simulink model "SAcell"  (R2023b)
settings: Solver=ode1  StartTime=0.0  StopTime=5000  FixedStep=0.1  RelTol=1e-3  EnableMultiTasking=on
model workspace: external: MAT-File SA.mat (data not in the file)
values from neighbouring files (symbols this model uses):
  bcl = 1500    [BH.mat]    (also in CN.mat; SA.mat = 814)
  erp = 108    [BH.mat]    (also in CN.mat = 214; SA.mat = 161.5)
  f = 0    [BH.mat]    (also in CN.mat = 0.8; SA.mat = 0.1)
  h = 0    [BH.mat]    (also in CN.mat = 0.2; Plottrace.m = gca; SA.mat = 0.2; plotCells.m = gca)
  hr = 0.1    [BH.mat]    (also in CN.mat; SA.mat)
  hs = 35    [BH.mat]    (also in CN.mat; SA.mat)
  j = 2    [BH.mat]    (also in CN.mat = 0; SA.mat = 0)
  m = 1    [BH.mat]    (also in CN.mat; SA.mat; plotCells.m; plotCells_second.m)
  r = 0.5    [BH.mat]    (also in CN.mat; SA.mat)
  s = 5    [BH.mat]    (also in CN.mat; SA.mat; plotCells.m = [4 8 9 10 11]; plotCells_second.m = [4 8 9 10 11])
  Vh = -15    [BH.mat]    (also in CN.mat = -4; SA.mat = -4)
libraries: Libs x1
settings Model: PauseTimes=18000  Creator=wai484  LastModifiedBy=wai484
settings SolverCC: AlgebraicLoopSolver=TrustRegion
settings DataIOCC: LimitDataPoints=on  SaveFormat=Array  ReturnWorkspaceOutputs=off
settings OptimizationCC: LifeSpan=inf
settings DebuggingCC: SolverPrmCheckMsg=warning  UnconnectedInputMsg=warning  UnconnectedOutputMsg=warning  UnconnectedLineMsg=warning  SFUnexpectedBacktrackingDiag=warning  SFNoUnconditionalDefaultTransitionDiag=warning  SFExecutionAtInitializationDiag=none  ArithmeticOperatorsInVariantConditions=warning
settings HardwareCC: ProdBitPerPointer=32  ProdBitPerSizeT=32  ProdBitPerPtrDiffT=32  ProdLargestAtomicFloat=None  ProdIntDivRoundTo=Undefined  ProdEndianess=Unspecified  ProdWordSize=32  ProdHWDeviceType=32-bit Generic
settings ModelReferenceCC: EnableRefExpFcnMdlSchedulingChecks=on  PropagateSignalLabelsOutOfModel=off
settings SFSimCC: SimUseLocalCustomCode=off  CustomCodeUndefinedFunction=UseInterfaceOnly
settings RTWCC: RTWUseLocalCustomCode=off
settings CodeAppCC: StateflowObjectComments=on
settings GRTTargetCC: TargetLangStandard=C89/C90 (ANSI)
settings ConfigComp: CovMetricSettings=dw  CovSaveCumulativeToWorkspaceVar=on  CovSaveSingleToWorkspaceVar=on  CovExternalEMLEnable=off  CovSFcnEnable=off

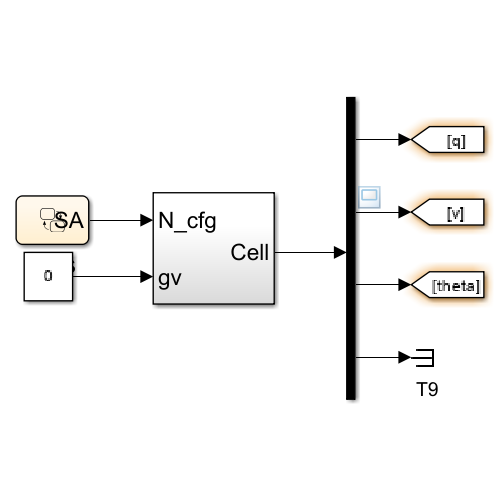
[thumbnail: Simulink's stored preview of the top-level diagram]
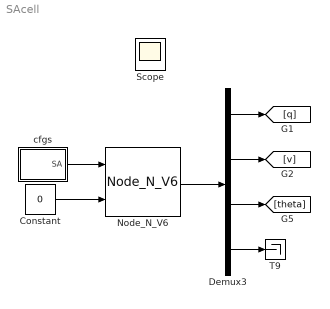
== system SAcell ==
  Constant : Constant  Value=0
  Demux3 : Demux  Outputs=[1, 1, 1,2]
  Node_N_V6 : Libs/Node_N_V6  SystemSampleTime=-1  VariantActivationTime=update diagram  AllowFlexibleInterface=on  Latency=0  AutoFrameSizeCalculation=off
  T9 : Terminator
  cfgs : Stateflow chart  TreatAsAtomicUnit=on
  Scope : Scope
  wires:
  Node_N_V6/1 -> Demux3/1
  Demux3/4 -> T9/1
  Demux3/1 -> [q]
  Demux3/2 -> [v]
  Demux3/3 -> [theta]
  Constant/1 -> Node_N_V6/2
  cfgs/1(SA) -> Node_N_V6/1

== stateflow chart SAcell/cfgs ==
  settings: executeAtInitialization=1
  state Ini
  (default) -> Ini : {SA=auto;}
  data: erp parameter; Vh parameter; hr parameter; hs parameter; m parameter; s parameter; j parameter; h parameter; f parameter; r parameter; bcl parameter; cfg function_output; SA output
  function cfg = auto:
    | function cfg = auto
    | 
    | BCL=bcl;
    | SD=2;
    | f1=0.1;
    | f2=0.25;
    | sigma1sq=0.0035;
    | sigma2sq=0.007;
    | 
    | d2=1.2810; 
    | erp_out=erp;
    | d0=-0.7732; 
    | MDP=-85.3;
    | VT=23.81; 
    | VR=47.94; 
    | Vh_out=Vh;
    | 
    | hr_out=hr; 
    | hs_out=hs;
    | s_out=s;
    | j_out=j;
    | m_out=m; 
    | 
    | h_out=h;
    | f_out=f;
    | 
    | r_out=r;
    | 
    | x=135.5;
    | y=295.5;
    | 
    | cfg=[BCL, SD, f1,f2,sigma1sq, sigma2sq,d2,erp_out,d0,MDP,VT,VR,Vh_out,hr_out,hs_out,s_out,j_out,m_out,h_out,f_out,r_out,x,y];
    | 
    | end
